simulink model "LLC_fullBridge"  (R2024a)
settings: Solver=ode23tb  StartTime=0.0  StopTime=0.1  RelTol=1e-3
undefined symbols (not defined in the file): Cr, fsw, Lm, Lr, n, P, Vin, Vo
libraries: spsCurrentMeasurementLib x7, spsSeriesRLCBranchLib x5, spsVoltageMeasurementLib x5, spsDiodeLib x4, spsMosfetLib x4, spsDCVoltageSourceLib x1, spsLinearTransformerLib x1, spsMeanLib x1, spspowerguiLib x1
settings Model: Creator=X-level  LastModifiedBy=X-level

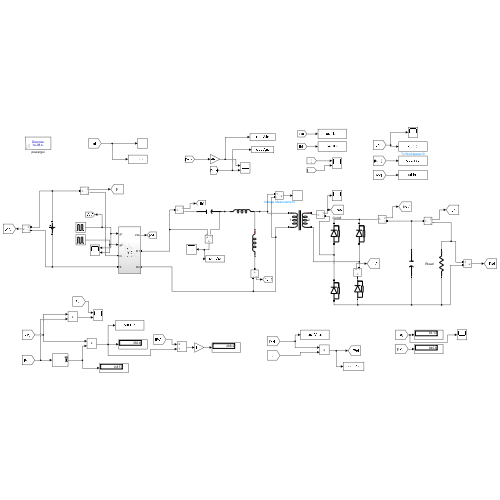
[thumbnail: Simulink's stored preview of the top-level diagram]
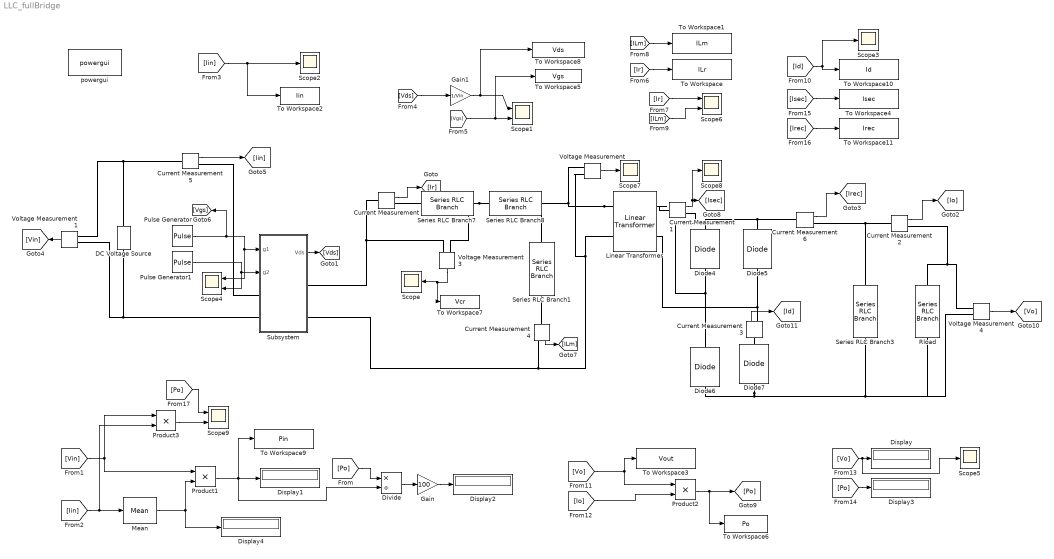
== system LLC_fullBridge ==
  Current Measurement{,1..6} (7 alike) : spsCurrentMeasurementLib/Current Measurement  PhasorSimulation=off  OutputType=Complex  PSBequivalent=0
  DC Voltage Source : spsDCVoltageSourceLib/DC Voltage Source  Amplitude=Vin  Measurements=None
  Diode{4..7} (4 alike) : spsDiodeLib/Diode  Ron=0.001  Lon=0  Vf=0.8  IC=0  UseSnubber=0  Rs=500  Cs=250e-9  Measurements=off
  Display{,1..4} (5 alike) : Display
  Divide : Product  Inputs=*/
  Gain : Gain  Gain=100
  Gain1 : Gain  Gain=1/Vin
  Linear Transformer : spsLinearTransformerLib/Linear Transformer  UNITS=SI  NominalPower=[P 100e3 ]  winding1=n*[1 0.001 1e-08]  winding2=1*[1 0.001 1e-08]  ThreeWindings=off  winding3=[3.15e+05 7.35e+05 46.792]  RmLm=[1e6 500]  Measurements=None  DataType=on
  Mean : spsMeanLib/Mean  Freq=fsw  Vinit=10  Ts=0
  Product1 : Product
  Product2 : Product
  Product3 : Product
  Pulse Generator : DiscretePulseGenerator  PulseType=Time based  Period=1/fsw  PulseWidth=49.1
  Pulse Generator1 : DiscretePulseGenerator  PulseType=Time based  Period=1/fsw  PulseWidth=49.1  PhaseDelay=0.5*(1/fsw)
  Rload : spsSeriesRLCBranchLib/Series RLC Branch  LConnTagsString=__new0  RConnTagsString=__new0  BranchType=R  Resistance=Vo*Vo/P  Inductance=1e-3  SetiL0=off  InitialCurrent=0  Capacitance=100e-6  Setx0=off  InitialVoltage=0  Measurements=None
  Scope{,2..3,5,7..8} (6 alike) : Scope
  Scope{1,4,6,9} (4 alike) : Scope  NumInputPorts=2
  Series RLC Branch1 : spsSeriesRLCBranchLib/Series RLC Branch  LConnTagsString=__new0  RConnTagsString=__new0  BranchType=L  Resistance=1  Inductance=Lm  SetiL0=off  InitialCurrent=0  Capacitance=1e-6  Setx0=off  InitialVoltage=0  Measurements=None
  Series RLC Branch3 : spsSeriesRLCBranchLib/Series RLC Branch  LConnTagsString=__new0  RConnTagsString=__new0  BranchType=C  Resistance=1  Inductance=1e-3  SetiL0=off  InitialCurrent=0  Capacitance=1000e-6  Setx0=off  InitialVoltage=0  Measurements=None
  Series RLC Branch7 : spsSeriesRLCBranchLib/Series RLC Branch  LConnTagsString=__new0  RConnTagsString=__new0  BranchType=C  Resistance=1  Inductance=1e-3  SetiL0=off  InitialCurrent=0  Capacitance=Cr  Setx0=off  InitialVoltage=0  Measurements=None
  Series RLC Branch8 : spsSeriesRLCBranchLib/Series RLC Branch  LConnTagsString=__new0  RConnTagsString=__new0  BranchType=L  Resistance=1  Inductance=Lr  SetiL0=off  InitialCurrent=0  Capacitance=1e-6  Setx0=off  InitialVoltage=0  Measurements=None
  Subsystem : Subsystem
  To Workspace : ToWorkspace  VariableName=ILr  SampleTime=-1
  To Workspace1 : ToWorkspace  VariableName=ILm  SampleTime=-1
  To Workspace10 : ToWorkspace  VariableName=Id  SampleTime=-1
  To Workspace11 : ToWorkspace  VariableName=Irec  SampleTime=-1
  To Workspace2 : ToWorkspace  VariableName=Iin  SampleTime=-1
  To Workspace3 : ToWorkspace  VariableName=Vout  SampleTime=-1
  To Workspace4 : ToWorkspace  VariableName=Isec  SampleTime=-1
  To Workspace5 : ToWorkspace  VariableName=Vgs  SampleTime=-1
  To Workspace6 : ToWorkspace  VariableName=Po  SampleTime=-1
  To Workspace7 : ToWorkspace  VariableName=Vcr  SampleTime=-1
  To Workspace8 : ToWorkspace  VariableName=Vds  SampleTime=-1
  To Workspace9 : ToWorkspace  VariableName=Pin  SampleTime=-1
  Voltage Measurement{,1,3..4} (4 alike) : spsVoltageMeasurementLib/Voltage Measurement  PhasorSimulation=off  OutputType=Complex  PSBequivalent=0
  powergui : spspowerguiLib/powergui  Priority=1  SimulationMode=Discrete  SampleTime=1e-8  frequency=60  Iterations=50  frequencyindice=0  Pbase=100e6  ErrMax=1e-4  UnitsV=kV  UnitsW=MW  buscounter=0  FunctionMessages=off  echomessages=off  EnableUseOfTLC=off  CurrentSourceSwitches=off  DisableSnubberDevices=off  DisableRonSwitches=off  DisableVfSwitches=off  DisplayEquations=off  AutomaticDiscreteSolvers=off  SolverType=Tustin/Backward Euler (TBE)  Interpol=off  ExternalGateDelay=off  methode=off  Ts=100  x0status=blocks  SPID=on  SwTol=0  HookPort=off  NonlinearTolerance=1e-4  nMaxIteration=100  ContinueOnMaxIteration=off  RestoreLinks=warning  ResistiveCurrentMeasurement=off  Frange=[0:2:500]  Ylog=off  Xlog=on  ShowGrid=off  save=off  variable=ZData  structure=0  ZoomFFT=off  StartTime=0.0  cycles=1  DisplayStyle=1  fundamental=60  FreqAxis=off  MaxFrequency=1000  frequencyindicesteady=1  RmsSteady=1  display=off
  wires:
  Voltage Measurement4/1 -> [Vo]
  Gain1/1 -> Scope1/1, To Workspace8/1
  Divide/1 -> Gain/1
  Product1/1 -> Display1/1, To Workspace9/1, Divide/2
  Current Measurement2/1 -> [Io]
  Current Measurement/1 -> [Ir]
  Gain/1 -> Display2/1
  Voltage Measurement3/1 -> Scope/1, To Workspace7/1
  Voltage Measurement/1 -> Scope7/1
  [Po] -> Divide/1
  Pulse Generator/1 -> Scope4/1, Subsystem/1(g1), [Vgs]
  Pulse Generator1/1 -> Subsystem/2(g2), Scope4/2
  Voltage Measurement1/1 -> [Vin]
  [Vin] -> Product3/1, Product1/1
  Current Measurement5/1 -> [Iin]
  [Iin] -> Product3/2, Mean/1
  [Iin] -> To Workspace2/1, Scope2/1
  Subsystem/1(Vds) -> [Vds]
  [Vds] -> Gain1/1
  [Vgs] -> To Workspace5/1, Scope1/2
  [Ir] -> To Workspace/1
  [Ir] -> Scope6/1
  Current Measurement4/1 -> [ILm]
  [ILm] -> To Workspace1/1
  [ILm] -> Scope6/2
  [Id] -> To Workspace10/1, Scope3/1
  [Vo] -> Product2/1, To Workspace3/1
  Product2/1 -> To Workspace6/1, [Po]
  [Io] -> Product2/2
  Current Measurement1/1 -> Scope8/1, [Isec]
  [Vo] -> Scope5/1, Display/1
  [Po] -> Display3/1
  Mean/1 -> Display4/1, Product1/2
  Product3/1 -> Scope9/2
  Current Measurement3/1 -> [Id]
  [Isec] -> To Workspace4/1
  Current Measurement6/1 -> [Irec]
  [Irec] -> To Workspace11/1
  [Po] -> Scope9/1
  connections:
  Diode5/RConn1 -- Diode4/RConn1 -- Current Measurement6/LConn1
  Diode4/LConn1 -- Diode6/RConn1 -- Current Measurement1/RConn1
  Diode5/LConn1 -- Current Measurement3/RConn1 -- Linear Transformer/RConn2
  Linear Transformer/LConn1 -- Series RLC Branch1/LConn1 -- Series RLC Branch8/RConn1 -- Voltage Measurement/LConn1
  Current Measurement2/RConn1 -- Rload/LConn1 -- Voltage Measurement4/LConn1
  Diode7/LConn1 -- Voltage Measurement4/LConn2 -- Rload/RConn1 -- Series RLC Branch3/RConn1 -- Diode6/LConn1
  Linear Transformer/RConn1 -- Current Measurement1/LConn1
  Current Measurement4/LConn1 -- Series RLC Branch1/RConn1
  Current Measurement/RConn1 -- Series RLC Branch7/LConn1
  Series RLC Branch8/LConn1 -- Series RLC Branch7/RConn1 -- Voltage Measurement3/LConn2
  DC Voltage Source/LConn1 -- Subsystem/LConn2 -- Voltage Measurement1/LConn2
  Voltage Measurement/LConn2 -- Linear Transformer/LConn2 -- Subsystem/RConn2 -- Current Measurement4/RConn1
  Voltage Measurement3/LConn1 -- Subsystem/RConn1 -- Current Measurement/LConn1
  Subsystem/LConn1 -- Current Measurement5/RConn1
  DC Voltage Source/RConn1 -- Voltage Measurement1/LConn1 -- Current Measurement5/LConn1
  Current Measurement3/LConn1 -- Diode7/RConn1
  Current Measurement2/LConn1 -- Current Measurement6/RConn1 -- Series RLC Branch3/LConn1

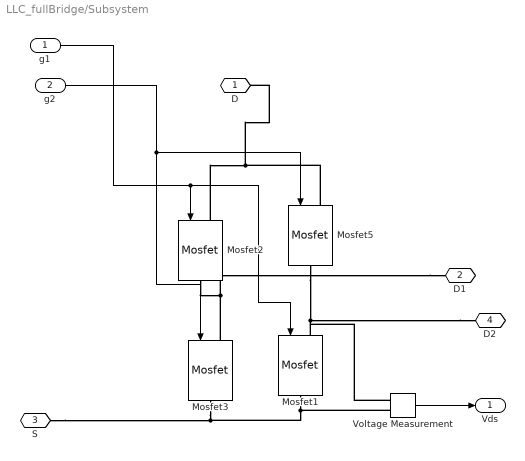
== system LLC_fullBridge/Subsystem ==
  g1 : Inport
  g2 : Inport  Port=2
  Mosfet{1..3,5} (4 alike) : spsMosfetLib/Mosfet  Ron=0.01  Lon=0  Rd=0.01  Vfd=0  IC=0  Rs=1e5  Cs=inf  Measurements=off
  Voltage Measurement : spsVoltageMeasurementLib/Voltage Measurement  PhasorSimulation=off  OutputType=Complex  PSBequivalent=0
  D : PMIOPort  Side=Left
  D1 : PMIOPort  Port=2  Side=Right
  S : PMIOPort  Port=3  Side=Left
  D2 : PMIOPort  Port=4  Side=Right
  Vds : Outport
  wires:
  g2/1 -> Mosfet3/1, Mosfet5/1
  g1/1 -> Mosfet1/1, Mosfet2/1
  Voltage Measurement/1 -> Vds/1
  connections:
  D1/RConn1 -- Mosfet3/LConn1 -- Mosfet2/RConn1
  D2/RConn1 -- Voltage Measurement/LConn1 -- Mosfet1/LConn1 -- Mosfet5/RConn1
  S/RConn1 -- Mosfet3/RConn1 -- Mosfet1/RConn1 -- Voltage Measurement/LConn2
  D/RConn1 -- Mosfet5/LConn1 -- Mosfet2/LConn1
